simulink model "simulate_model_operatingLoss_mode"  (R2026a)
settings: Solver=VariableStepAuto  StopTime=86400*10  FixedStep=60.0
values from neighbouring files (symbols this model uses):
  Ts = 60    [controller_setup_V2.m]
  u0 = [0.80; 150; 1.7; 0.50; 0.35; 0]    [controller_setup_V2.m]
  x0 = [0.92; 70; 0]    [controller_setup_V2.m]
  y0 = [0.92; 70; 0]    [controller_setup_V2.m]
undefined symbols (not defined in the file or in its folder): DiscIntNeverNeededParam
libraries: slident x6, mpclib x1, eeGeneralControl x1, eeStairGenerator x1
settings Model: Creator=dangs  LastModifiedBy=dangs
settings DebuggingCC: InheritedTsInSrcMsg=none

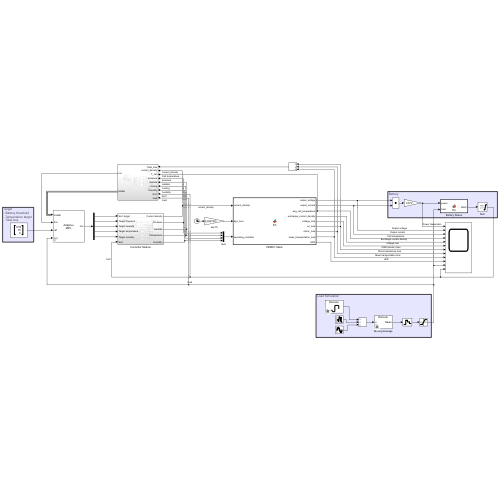
[thumbnail: Simulink's stored preview of the top-level diagram]
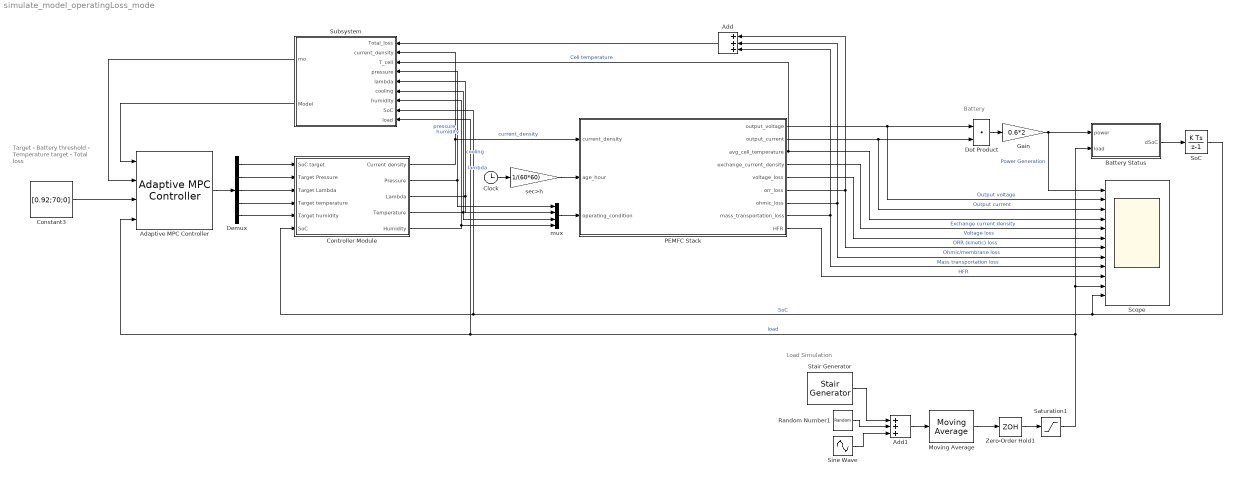
== system simulate_model_operatingLoss_mode ==
  note: Target
      | - Battery threshold
      | - Temperature target
      | - Total loss
  note: Battery
  note: Load Simulation
  Adaptive MPC Controller : mpclib/Adaptive MPC Controller  SCDEnableBlockLinearizationSpecification=on  mpcobj=mpcobj  enable_value=0  updateMPCinCallerWorkspace=on  md_inport=on  mv_inport=off  uref_inport=off  return_cost=off  return_mvseq=off  return_qpstatus=off  return_xseq=off  return_state=off  return_ovseq=off  state_inport=off  isltv_plant=off  umin_inport=off  umax_inport=off  ymin_inport=off  ymax_inport=off  cc_inport=off  ywt_inport=off  uwt_inport=off  duwt_inport=off  rhoeps_inport=off  pm_inport=off  MaximumP=10  HorizonChoice=FixedHorizon  BlockDataType=double  SampleTimeInherited=off  switch_inport=off
  Add : Sum  Inputs=+++
  Add1 : Sum  Inputs=+++
  Battery Status : MATLAB Function  TreatAsAtomicUnit=on
  Clock : Clock
  Constant3 : Constant  Value=[0.92;70;0]  VectorParams1D=off
  Controller Module : Subsystem
  Demux : Demux  Outputs=5
  Dot Product : DotProduct  OutDataTypeStr=Inherit: Inherit via internal rule
  Gain : Gain  Gain=0.6*2
  Moving Average : eeGeneralControl/Moving Average  VariantControl=Variant1  LabelModeActiveChoice=Discrete  f=60  x0=0  BufferSize=8192  Ts=Ts
      settings: LibrarySourceBlock=ee_sl_lib/General Control/Moving Average
  PEMFC Stack : MATLAB Function  TreatAsAtomicUnit=on
  Random Number1 : RandomNumber  Mean=1000  Variance=1000  SampleTime=Ts
  Saturation1 : Saturate  UpperLimit=inf  LowerLimit=0
  Scope : Scope  NumInputPorts=12
      settings: ActiveDisplayYMinimum=-4588.6379394869737  ActiveDisplayYMaximum=41297.741455382769
  Sine Wave : Sin  Amplitude=3500  Bias=30500  Frequency=2*pi/86400  Phase=-pi/2  SampleTime=Ts
  SoC : DiscreteIntegrator  InitialCondition=0.3  SampleTime=Ts  LimitOutput=on  UpperSaturationLimit=1  LowerSaturationLimit=0  ICPrevOutput=DiscIntNeverNeededParam  ICPrevScaledInput=DiscIntNeverNeededParam
  Stair Generator : eeStairGenerator/Stair Generator  LabelModeActiveChoice=Discrete  TimeInput=[0.3 0.5 0.7 1]*86400  AmplitudeInput=[666.67,333.33,1800,1000]  SampleTime=-1  RepeatPattern=on  OutDataTypeStr=double
      settings: LibrarySourceBlock=ee_sl_lib/General Control/Stair Generator
  Subsystem : Subsystem
  Zero-Order Hold1 : ZeroOrderHold  SampleTime=Ts
  mux : Mux
  sec>h : Gain  Gain=1/(60*60)
  wires:
  Clock/1 -> sec>h/1
  sec>h/1 -> PEMFC Stack/2(age_hour)
  Demux/1 -> Controller Module/1(SoC target)
  Demux/2 -> Controller Module/2(Target Pressure)
  Demux/3 -> Controller Module/3(Target Lambda)
  Demux/4 -> Controller Module/4(Target temperature)
  Demux/5 -> Controller Module/5(Target humidity)
  Controller Module/1(Current density) -> Subsystem/2(current_density), PEMFC Stack/1(current_density)  "current_density"
  Adaptive MPC Controller/1 -> Demux/1
  Controller Module/2(Pressure) -> Subsystem/4(pressure), mux/1  "pressure"
  Controller Module/3(Lambda) -> mux/2, Subsystem/5(lambda)  "lambda"
  Controller Module/4(Temperature) -> mux/3, Subsystem/6(cooling)  "cooling"
  Controller Module/5(Humidity) -> mux/4, Subsystem/7(humidity)  "humidity"
  mux/1 -> PEMFC Stack/3(operating_condition)
  Battery Status/1(dSoC) -> SoC/1
  Constant3/1 -> Adaptive MPC Controller/3
  Gain/1 -> Battery Status/1(power), Scope/1  "Power Generation"
  Saturation1/1 -> Subsystem/9(load), Adaptive MPC Controller/4, Scope/11, Battery Status/2(load)  "load"
  SoC/1 -> Subsystem/8(SoC), Controller Module/6(SoC), Scope/12  "SoC"
  Dot Product/1 -> Gain/1
  PEMFC Stack/2(output_current) -> Scope/3, Dot Product/2  "Output current"
  PEMFC Stack/1(output_voltage) -> Scope/2, Dot Product/1  "Output voltage"
  PEMFC Stack/3(avg_cell_temperature) -> Scope/4, Subsystem/3(T_cell)  "Cell temperature"
  PEMFC Stack/4(exchange_current_density) -> Scope/5  "Exchange current density"
  PEMFC Stack/5(voltage_loss) -> Scope/6  "Voltage loss"
  PEMFC Stack/6(orr_loss) -> Add/1, Scope/7  "ORR (kinetic) loss"
  PEMFC Stack/7(ohmic_loss) -> Add/2, Scope/8  "Ohmic/membrane loss"
  PEMFC Stack/8(mass_transportation_loss) -> Add/3, Scope/9  "Mass transportation loss"
  PEMFC Stack/9(HFR) -> Scope/10  "HFR"
  Subsystem/2(Model) -> Adaptive MPC Controller/1
  Subsystem/1(mo) -> Adaptive MPC Controller/2
  Zero-Order Hold1/1 -> Saturation1/1
  Add1/1 -> Moving Average/1
  Random Number1/1 -> Add1/2
  Sine Wave/1 -> Add1/3
  Moving Average/1 -> Zero-Order Hold1/1
  Stair Generator/1 -> Add1/1
  Add/1 -> Subsystem/1(Total_loss)

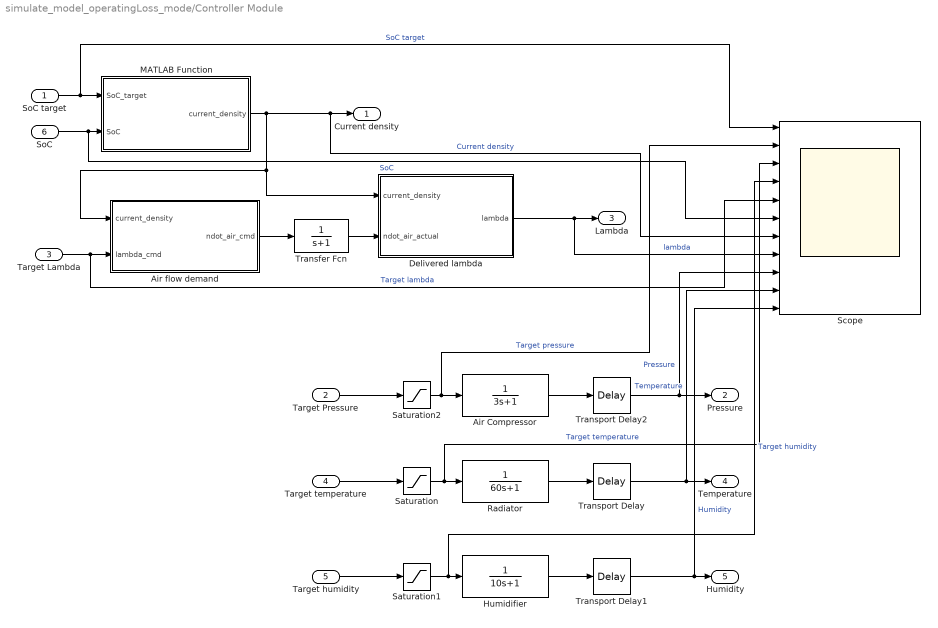
== system simulate_model_operatingLoss_mode/Controller Module ==
  SoC target : Inport
  Target Pressure : Inport  Port=2
  Target Lambda : Inport  Port=3
  Target temperature : Inport  Port=4
  Target humidity : Inport  Port=5
  SoC : Inport  Port=6
  Air Compressor : TransferFcn  Denominator=[3 1]
  Air flow demand : MATLAB Function  TreatAsAtomicUnit=on
  Delivered lambda : MATLAB Function  TreatAsAtomicUnit=on
  Humidifier : TransferFcn  Denominator=[10 1]
  MATLAB Function : MATLAB Function  TreatAsAtomicUnit=on
  Radiator : TransferFcn  Denominator=[60 1]
  Saturation : Saturate  UpperLimit=75  LowerLimit=55
  Saturation1 : Saturate  UpperLimit=0.9  LowerLimit=0.3
  Saturation2 : Saturate  UpperLimit=200  LowerLimit=50
  Scope : Scope  NumInputPorts=11
      settings: ActiveDisplayYMinimum=0.70000000000000007  ActiveDisplayYMaximum=0.9
  Transfer Fcn : TransferFcn  Denominator=[1 1]
  Transport Delay : TransportDelay  DelayTime=10
  Transport Delay1 : TransportDelay  DelayTime=3
  Transport Delay2 : TransportDelay  DelayTime=0.5
  Current density : Outport
  Pressure : Outport  Port=2
  Lambda : Outport  Port=3
  Temperature : Outport  Port=4
  Humidity : Outport  Port=5
  wires:
  Humidifier/1 -> Transport Delay1/1
  Transport Delay2/1 -> Scope/9, Pressure/1  "Pressure"
  Saturation2/1 -> Scope/2, Air Compressor/1  "Target pressure"
  Transport Delay1/1 -> Scope/11, Humidity/1  "Humidity"
  Air flow demand/1(ndot_air_cmd) -> Transfer Fcn/1
  Transfer Fcn/1 -> Delivered lambda/2(ndot_air_actual)
  Delivered lambda/1(lambda) -> Scope/8, Lambda/1  "lambda"
  MATLAB Function/1(current_density) -> Scope/7, Current density/1, Delivered lambda/1(current_density), Air flow demand/1(current_density)  "Current density"
  Target Pressure/1 -> Saturation2/1
  Air Compressor/1 -> Transport Delay2/1
  SoC target/1 -> Scope/1, MATLAB Function/1(SoC_target)  "SoC target"
  Saturation1/1 -> Scope/4, Humidifier/1  "Target humidity"
  Saturation/1 -> Scope/3, Radiator/1  "Target temperature"
  Radiator/1 -> Transport Delay/1
  Transport Delay/1 -> Scope/10, Temperature/1  "Temperature"
  Target Lambda/1 -> Scope/5, Air flow demand/2(lambda_cmd)  "Target lambda"
  Target temperature/1 -> Saturation/1
  Target humidity/1 -> Saturation1/1
  SoC/1 -> Scope/6, MATLAB Function/2(SoC)  "SoC"

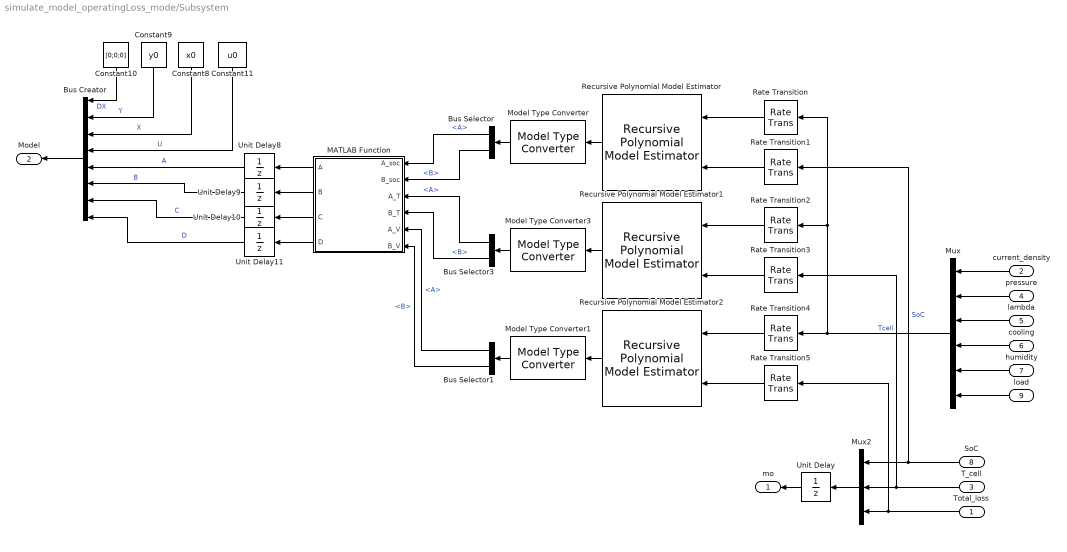
== system simulate_model_operatingLoss_mode/Subsystem ==
  Total_loss : Inport
  current_density : Inport  Port=2
  T_cell : Inport  Port=3
  pressure : Inport  Port=4
  lambda : Inport  Port=5
  cooling : Inport  Port=6
  humidity : Inport  Port=7
  SoC : Inport  Port=8
  load : Inport  Port=9
  Bus Creator : BusCreator  Inputs=8
  Bus Selector : BusSelector  OutputSignals=A,B
  Bus Selector1 : BusSelector  OutputSignals=A,B
  Bus Selector3 : BusSelector  OutputSignals=A,B
  Constant10 : Constant  Value=[0;0;0]  VectorParams1D=off
  Constant11 : Constant  Value=u0  VectorParams1D=off
  Constant8 : Constant  Value=x0  VectorParams1D=off
  Constant9 : Constant  Value=y0  VectorParams1D=off
  MATLAB Function : MATLAB Function  TreatAsAtomicUnit=on
  Model Type Converter : slident/Estimators/Model Type Converter  InputModelType=ARX
  Model Type Converter1 : slident/Estimators/Model Type Converter  InputModelType=ARX
  Model Type Converter3 : slident/Estimators/Model Type Converter  InputModelType=ARX
  Mux : Mux  Inputs=6
  Mux2 : Mux  Inputs=3
  Rate Transition{,1..5} (6 alike) : RateTransition
  Recursive Polynomial Model Estimator : slident/Estimators/Recursive Polynomial Model Estimator  ModelStructure=ARX  InitialEstimateSource=None  A0=na  B0=nb  C0=1  D0=1  F0=1  nk=nk  P0=1e2  InitialInputs=0  InitialOutputs=0  History=Infinite  WindowLength=200  EstimationMethod=Forgetting Factor  AdaptationParameter=0.95  HasTimeVaryingAdaptationParameter=off  NormalizationBias=eps  OutputError=off  OutputP=off  AddEnablePort=off  InputProcessing=Sample-based  Ts=Ts
  Recursive Polynomial Model Estimator1 : slident/Estimators/Recursive Polynomial Model Estimator  ModelStructure=ARX  InitialEstimateSource=None  A0=na  B0=nb  C0=1  D0=1  F0=1  nk=nk  P0=1e2  InitialInputs=0  InitialOutputs=0  History=Infinite  WindowLength=200  EstimationMethod=Forgetting Factor  AdaptationParameter=0.95  HasTimeVaryingAdaptationParameter=off  NormalizationBias=eps  OutputError=off  OutputP=off  AddEnablePort=off  InputProcessing=Sample-based  Ts=Ts
  Recursive Polynomial Model Estimator2 : slident/Estimators/Recursive Polynomial Model Estimator  ModelStructure=ARX  InitialEstimateSource=None  A0=na  B0=nb  C0=1  D0=1  F0=1  nk=nk  P0=1e2  InitialInputs=0  InitialOutputs=0  History=Infinite  WindowLength=200  EstimationMethod=Forgetting Factor  AdaptationParameter=0.95  HasTimeVaryingAdaptationParameter=off  NormalizationBias=eps  OutputError=off  OutputP=off  AddEnablePort=off  InputProcessing=Sample-based  Ts=Ts
  Unit Delay{,8..11} (5 alike) : UnitDelay  SampleTime=Ts
  mo : Outport
  Model : Outport  Port=2
  wires:
  current_density/1 -> Mux/1
  cooling/1 -> Mux/4
  load/1 -> Mux/6
  Rate Transition1/1 -> Recursive Polynomial Model Estimator/2
  SoC/1 -> Mux2/1, Rate Transition1/1  "SoC"
  Mux/1 -> Rate Transition2/1, Rate Transition/1, Rate Transition4/1
  Rate Transition/1 -> Recursive Polynomial Model Estimator/1
  lambda/1 -> Mux/3
  pressure/1 -> Mux/2
  humidity/1 -> Mux/5
  T_cell/1 -> Rate Transition3/1, Mux2/2  "Tcell"
  Rate Transition2/1 -> Recursive Polynomial Model Estimator1/1
  Rate Transition3/1 -> Recursive Polynomial Model Estimator1/2
  Rate Transition5/1 -> Recursive Polynomial Model Estimator2/2
  Rate Transition4/1 -> Recursive Polynomial Model Estimator2/1
  MATLAB Function/1(A) -> Unit Delay8/1
  MATLAB Function/4(D) -> Unit Delay11/1
  MATLAB Function/3(C) -> Unit Delay10/1
  MATLAB Function/2(B) -> Unit Delay9/1
  Constant10/1 -> Bus Creator/1  "DX"
  Constant9/1 -> Bus Creator/2  "Y"
  Constant8/1 -> Bus Creator/3  "X"
  Constant11/1 -> Bus Creator/4  "U"
  Unit Delay8/1 -> Bus Creator/5  "A"
  Unit Delay9/1 -> Bus Creator/6  "B"
  Unit Delay10/1 -> Bus Creator/7  "C"
  Unit Delay11/1 -> Bus Creator/8  "D"
  Bus Creator/1 -> Model/1
  Recursive Polynomial Model Estimator/1 -> Model Type Converter/1
  Model Type Converter/1 -> Bus Selector/1
  Bus Selector/1 -> MATLAB Function/1(A_soc)  "<A>"
  Bus Selector/2 -> MATLAB Function/2(B_soc)  "<B>"
  Model Type Converter3/1 -> Bus Selector3/1
  Recursive Polynomial Model Estimator1/1 -> Model Type Converter3/1
  Model Type Converter1/1 -> Bus Selector1/1
  Recursive Polynomial Model Estimator2/1 -> Model Type Converter1/1
  Bus Selector3/1 -> MATLAB Function/3(A_T)  "<A>"
  Bus Selector3/2 -> MATLAB Function/4(B_T)  "<B>"
  Bus Selector1/1 -> MATLAB Function/5(A_V)  "<A>"
  Bus Selector1/2 -> MATLAB Function/6(B_V)  "<B>"
  Total_loss/1 -> Rate Transition5/1, Mux2/3
  Unit Delay/1 -> mo/1
  Mux2/1 -> Unit Delay/1

== matlab function simulate_model_operatingLoss_mode/Controller Module/Air flow demand ==
  data: current_density input; lambda_cmd input; ndot_air_cmd output
function ndot_air_cmd = fcn(current_density, lambda_cmd)
    % Air molar flow needed to hold lambda_cmd at the present current, with a
    % compressor minimum-flow floor (from the durability log, ~84 A equivalent).
    N = 10; A = 280; F = 96485; O2frac = 0.2095;
    I = current_density * A; % stack current [A]
    I_min = 10;
    ndot_stoich = N * I / (4*F) / O2frac; % air for lambda = 1 at this current
    ndot_stoich_min = N * I_min / (4*F) / O2frac;
    ndot_air_cmd = lambda_cmd * max(ndot_stoich, ndot_stoich_min);   % [mol/s]
end

== matlab function simulate_model_operatingLoss_mode/PEMFC Stack ==
  data: current_density input; age_hour input; operating_condition input; output_voltage output; output_current output; avg_cell_temperature output; exchange_current_density output; voltage_loss output; orr_loss output; ohmic_loss output; mass_transportation_loss output; HFR output
function [output_voltage, output_current,  avg_cell_temperature, ...
          exchange_current_density, voltage_loss, orr_loss, ohmic_loss, ...
          mass_transportation_loss, HFR] = fcn(current_density, age_hour, operating_condition)
    % Consolidated PEMFC degradation / voltage model for a 10-cell stack.
    % Per-cell losses/temperature/HFR/j0 with 10-cell stack voltage and current.
    %
    % INPUTS
    %   current_density      j      [A/cm^2]  (default: 0.5)
    %   age_hour             t      [h]       (default: 0)
    %   operating_condition  1x4 = [p_c (kPaG), lambda_c, T_in (degC), RH_c]
    %                                         (default: [150, 1.7, 70, 0.35])
    %
    % OUTPUTS
    %   output_voltage             10 * cell_voltage [V]
    %   output_current             280 * current_density * 10 [A] (280 cm^2, 10 cells)
    %   orr_loss                   per-cell activation (ORR) overpotential [V]
    %   ohmic_loss                 per-cell ohmic / membrane overpotential [V]
    %   mass_transportation_loss   per-cell mass-transport overpotential [V]
    %   avg_cell_temperature       mean cell temperature [degC]
    %   exchange_current_density   ORR exchange current density j0 [A/cm^2]
    %   voltage_loss               per-cell aging loss vs. BoL at same setpoint [mV]
    %   HFR                        high-frequency resistance [Ohm*cm^2]

    N_cells = 10;
    A_cell  = 280; % [cm^2]

    % unpack setpoint
    p_c  = operating_condition(1); % cathode outlet pressure [kPaG]
    lam  = operating_condition(2); % cathode stoichiometry [-]
    T_in = operating_condition(3); % coolant inlet temperature [degC]
    RH   = operating_condition(4); % cathode inlet relative humidity [-]

    % thermal-model coefficients [a, b_flow, c_j2, d_Tin, e_age]
    a = -0.3687; b = 1.6828; c = 0.2772; d = -0.0154; e = -0.1059;
    F_cl = 6.0; % coolant flow [L/min] (fixed)

    % mean cell temperature (semi-empirical thermal model)
    avg_cell_temperature = T_in + a + b.*current_density.*6./F_cl ...
                           + c.*current_density.^2 + d.*(T_in - 70) ...
                           + e.*age_hour./1000;

    % voltage + loss breakdown at this age
    [cell_voltage, orr_loss, ohmic_loss, mass_transportation_loss, ...
     exchange_current_density, HFR] = cellmodel(current_density, age_hour, ...
                                                avg_cell_temperature, p_c, lam, T_in, RH);

    % voltage at BoL (age 0), same setpoint, for the aging loss
    T_bol = T_in + a + b.*current_density.*6./F_cl + c.*current_density.^2 + d.*(T_in - 70);
    U_bol = cellmodel(current_density, 0, T_bol, p_c, lam, T_in, RH);
    voltage_loss = U_bol - cell_voltage; % [V], it is in mV

    output_current = A_cell .* current_density .* N_cells; % [A]
    output_voltage = max(N_cells .* cell_voltage, 0); % [V]
end

function [U, act, ohm, mt, j0, HFR] = cellmodel(j, age_h, T_cell, p_c, lam, T_in, RH)
    % physical constants
    R = 8.314; F = 96485; P0 = 101.325; % J/mol/K, C/mol, kPa
    Ea = 80; jx = exp(-6); tau = 300; % kJ/mol, A/cm^2, h
    % fitted voltage-model coefficients
    lnj0 = -13.6563; j0f = -0.4934; j0s = 0.0801;
    alpha = 0.9740;  gam = 0.4081;  nu  = 0.1985;
    lnc  = -6.9859;  m   = 2.0241;  cf  = 0.0897; cs = 0.2336; kT = 0.0117;
    hb0  = 0.0483;   hb1 = 0.0018;  hb2 = 0.0038; % HFR = hb0 + hb1*age/1000 + hb2*j
    % secondary operating params (fixed)
    lam_a = 1.5; RH_a = 0.50; dpa = 10; % anode stoich, anode RH, anode-cathode p offset

    T = T_cell + 273.15; % K
    lam = max(lam, 1.001);
    pa  = p_c + dpa; % anode gauge pressure [kPaG]

    % water vapour partial pressures (RH referenced to coolant inlet)
    pw_c = RH   .* psat(T_in);
    pw_a = RH_a .* psat(T_in);

    % reactant partial pressures (log-mean O2 along the cathode channel) [kPa]
    pO2 = 0.2095 .* (p_c + P0 - pw_c) .* (1./lam) ./ (-log(1 - 1./lam));
    pH2 = 0.80   .* (pa  + P0 - pw_a) .* (1 - 1./(2.*lam_a));

    % age factors
    gf = 1 - exp(-age_h ./ tau);   gs = age_h ./ 1000;

    % Nernst potential
    E = 1.229 - 8.46e-4 .* (T - 298.15) + R.*T./(2.*F) .* log(pH2./P0 .* sqrt(pO2./P0));

    % activation (ORR): exchange current drops with age
    j0  = exp(lnj0 + j0f.*gf + j0s.*gs) .* exp(-Ea.*1e3./R .* (1./T - 1./343.15));
    act = R.*T./(alpha.*F) .* (log((j + jx)./j0) - gam.*log(pO2./P0));

    % ohmic / membrane: HFR rises linearly with age (imposed from EIS)
    HFR = hb0 + hb1.*age_h./1000 + hb2.*j;
    ohm = j .* HFR .* (RH./0.35).^(-nu);

    % mass transport: amplitude grows with age
    mt = exp(lnc) .* (1 + cf.*gf + cs.*gs) .* exp(-kT.*(T - 343.15)) .* (j ./ (pO2./P0)).^m;

    U = E - act - ohm - mt;
end

function p = psat(t)
    % Magnus formula, kPa, t in degC
    p = 0.61094 .* exp(17.625 .* t ./ (t + 243.04));
end

== matlab function simulate_model_operatingLoss_mode/Controller Module/Delivered lambda ==
  data: current_density input; ndot_air_actual input; lambda output
function lambda = fcn(current_density, ndot_air_actual)
    % Delivered O2 / O2 demanded by the current. Dips below the command when the
    % flow lags a current rise -> that dip IS the starvation behaviour.
    N = 10; A = 280; F = 96485; O2frac = 0.2095;
    I = current_density * A;
    nO2_consumed = N * I / (4*F);
    nO2_supplied = ndot_air_actual * O2frac;
    if nO2_consumed < 1e-9
        lambda = 3; % idle: large excess air
    else
        lambda = nO2_supplied / nO2_consumed;
    end
    lambda = min(max(lambda, 1.001), 3); % math floor; validated range is 1.6-2.1
end

== matlab function simulate_model_operatingLoss_mode/Controller Module/MATLAB Function ==
  data: SoC_target input; current_density output; SoC input
function current_density = fcn(SoC_target, SoC)
    j_max      = 1.8;
    taper_band = 0.1;
    SoC_err = SoC_target - SoC;
    if SoC_err <= 0
        current_density = 0;
    else
        frac = min(SoC_err / taper_band, 1);
        current_density = j_max * frac;
    end
    current_density = max(0, min(current_density, j_max));
end

== matlab function simulate_model_operatingLoss_mode/Subsystem/MATLAB Function ==
  data: A_soc input; B_soc input; A_T input; A output; B output; C output; D output; B_T input; A_V input; B_V input
function [A,B,C,D] = arx2ss_mimo(A_soc,B_soc, A_T,B_T, A_V,B_V)
    A = [A_soc, 0,   0;
         0,   A_T,   0;
         0,   0,   A_V];     % 3x3
    B = [B_soc;
         B_T;
         B_V];               % 3x6
    C = eye(3);              % 3x3
    D = zeros(3,6);          % 3x6
end

== matlab function simulate_model_operatingLoss_mode/Battery Status ==
  data: power input; dSoC output; load input
function dSoC = fcn(power, load)
    V_batt  = 48;  Q_Ah = 50;
    E_cap_J = V_batt * Q_Ah * 3600;     % [J]
    runoff  = 0.4e3;                    % drain [W]
    dSoC = (power - load - runoff) / E_cap_J;   % dSoC/dt
end
